simulink model "Proyecto"  (R2023a)
settings: Solver=ode15s  StartTime=0.0  StopTime=10.0  RelTol=1e-3
libraries: fl_lib x16, nesl_utility x6, slpidlib x1
settings Model: Creator=hp  LastModifiedBy=hp
settings DataIOCC: SaveFormat=Array  SaveOutput=off  SignalLogging=off  DSMLogging=off  ReturnWorkspaceOutputs=off  TimeSaveName=t
settings DebuggingCC: AlgebraicLoopMsg=none  MaxConsecutiveZCsMsg=none  ModelReferenceExtraNoncontSigs=none  OperatingPointInterfaceChecksumMismatchMsg=none

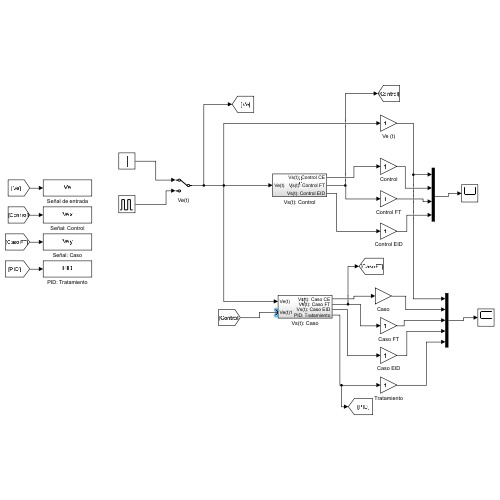
[thumbnail: Simulink's stored preview of the top-level diagram]
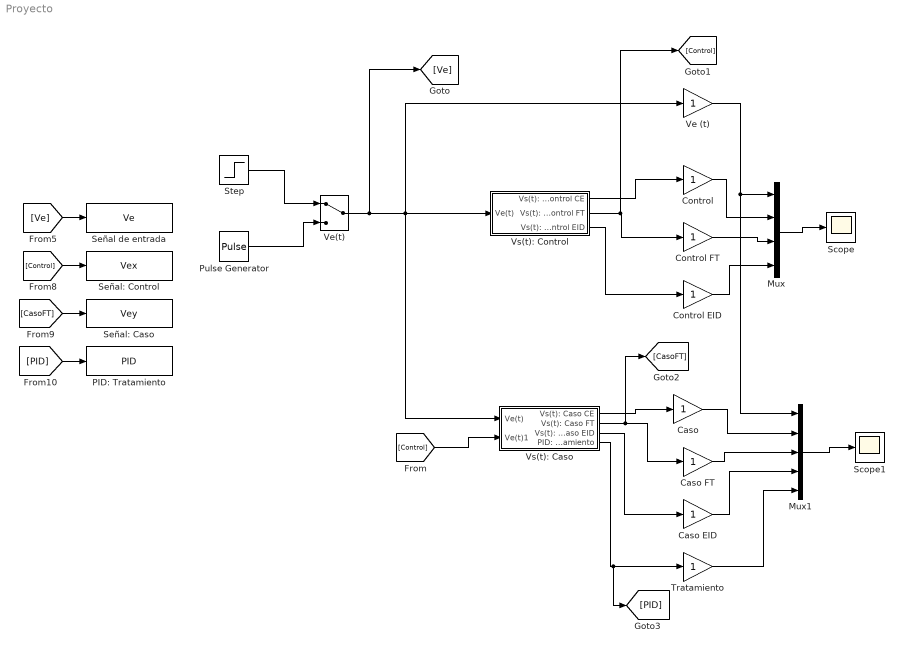
== system Proyecto ==
  Caso : Gain
  Caso EID : Gain
  Caso FT : Gain
  Control : Gain
  Control EID : Gain
  Control FT : Gain
  Mux : Mux
  Mux1 : Mux  Inputs=5
  PID: Tratamiento : ToWorkspace  VariableName=PID  SampleTime=-1
  Pulse Generator : DiscretePulseGenerator  PulseType=Time based  Period=10  PulseWidth=5
  Scope : Scope
  Scope1 : Scope
  Señal de entrada : ToWorkspace  VariableName=Ve  SampleTime=-1
  Señal: Caso : ToWorkspace  VariableName=Vey  SampleTime=-1
  Señal: Control : ToWorkspace  VariableName=Vex  SampleTime=-1
  Step : Step  SampleTime=0
  Tratamiento : Gain
  Ve (t) : Gain
  Ve(t) : ManualSwitch
  Vs(t): Caso : Subsystem
  Vs(t): Control : Subsystem
  wires:
  Step/1 -> Ve(t)/1
  Pulse Generator/1 -> Ve(t)/2
  Ve(t)/1 -> [Ve], Ve (t)/1, Vs(t): Caso/1(Ve(t)), Vs(t): Control/1(Ve(t))
  Mux/1 -> Scope/1
  Ve (t)/1 -> Mux1/1, Mux/1
  Vs(t): Control/1(Vs(t): Control CE) -> Control/1
  Control/1 -> Mux/2
  Vs(t): Caso/1(Vs(t): Caso CE) -> Caso/1
  Vs(t): Control/2(Vs(t): Control FT) -> [Control], Control FT/1
  Caso/1 -> Mux1/2
  Control FT/1 -> Mux/3
  Vs(t): Caso/2(Vs(t): Caso FT) -> [CasoFT], Caso FT/1
  Caso FT/1 -> Mux1/3
  Mux1/1 -> Scope1/1
  Vs(t): Control/3(Vs(t): Control EID) -> Control EID/1
  Control EID/1 -> Mux/4
  Vs(t): Caso/3(Vs(t): Caso EID) -> Caso EID/1
  Caso EID/1 -> Mux1/4
  [Control] -> Señal: Control/1
  [PID] -> PID: Tratamiento/1
  [CasoFT] -> Señal: Caso/1
  [Ve] -> Señal de entrada/1
  [Control] -> Vs(t): Caso/2(Ve(t)1)
  Vs(t): Caso/4(PID: Tratamiento) -> [PID], Tratamiento/1
  Tratamiento/1 -> Mux1/5

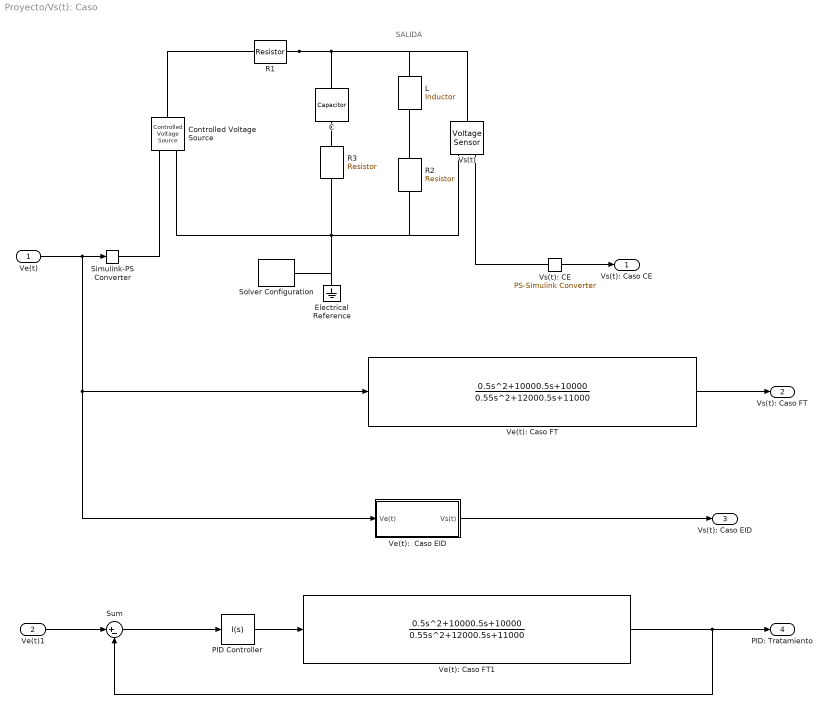
== system Proyecto/Vs(t): Caso ==
  note: SALIDA
  Ve(t) : Inport
  Ve(t)1 : Inport  Port=2
  C : fl_lib/Electrical/Electrical Elements/Capacitor  c=100e-6 F  r=1e-6 Ohm  g=0 1/Ohm  i_specify=off  i_priority=None  i=0 A  i_nominal_specify=off  i_nominal_unit=A  i_nominal_value=1  v_specify=off  v_priority=None  v=0 V  v_nominal_specify=off  v_nominal_unit=V  v_nominal_value=1  vc_specify=off  vc_priority=High  vc=0 V  vc_nominal_specify=off  vc_nominal_unit=V  vc_nominal_value=1
  Controlled Voltage Source : fl_lib/Electrical/Electrical Sources/Controlled Voltage Source
  Electrical Reference : fl_lib/Electrical/Electrical Elements/Electrical Reference
  L : fl_lib/Electrical/Electrical Elements/Inductor  l=500e-3 H  r=0 Ohm  g=1e-9 1/Ohm  i_specify=off  i_priority=None  i=0 A  i_nominal_specify=off  i_nominal_unit=A  i_nominal_value=1  v_specify=off  v_priority=None  v=0 V  v_nominal_specify=off  v_nominal_unit=V  v_nominal_value=1  i_L_specify=off  i_L_priority=High  i_L=0 A  i_L_nominal_specify=off  i_L_nominal_unit=A  i_L_nominal_value=1
  PID Controller : slpidlib/PID Controller  Controller=I  Form=Parallel  TimeDomain=Continuous-time  UseExternalTs=off  SampleTime=-1  IntegratorMethod=Forward Euler  FilterMethod=Forward Euler  ControllerParametersSource=internal  P=0  I=466.911552575517  UseKiTs=off  D=0  N=100  UseFilter=on  TunerSelectOption=Transfer Function Based (PID Tuner App)  InitialConditionSource=internal  InitialConditionForIntegrator=0  InitialConditionForFilter=0  DifferentiatorICPrevScaledInput=0  ExternalReset=none  TrackingMode=off  Kt=1  LimitOutput=off  SatLimitsSource=internal  UpperSaturationLimit=inf  LowerSaturationLimit=-inf  LinearizeAsGain=on  AntiWindupMode=none  Kb=1  LimitIntegrator=off  UpperIntegratorSaturationLimit=inf  LowerIntegratorSaturationLimit=-inf  POutMin=[]  POutMax=[]  IOutMin=[]  IOutMax=[]  DOutMin=[]  DOutMax=[]  NOutMin=[]  NOutMax=[]  SumOutMin=[]  SumOutMax=[]  SaturationOutMin=[]  SaturationOutMax=[]  PParamMin=[]  PParamMax=[]  IParamMin=[]  IParamMax=[]  DParamMin=[]  DParamMax=[]  NParamMin=[]  NParamMax=[]  KbParamMin=[]  KbParamMax=[]  KtParamMin=[]  KtParamMax=[]  KbOutMin=[]  KbOutMax=[]  KtOutMin=[]  KtOutMax=[]  IntegratorOutMin=[]  IntegratorOutMax=[]  FilterOutMin=[]  FilterOutMax=[]  SumI1OutMin=[]  SumI1OutMax=[]  SumI2OutMin=[]  SumI2OutMax=[]  SumI3OutMin=[]  SumI3OutMax=[]  SumI4OutMin=[]  SumI4OutMax=[]  SumDOutMin=[]  SumDOutMax=[]  DifferentiatorOutMin=[]  DifferentiatorOutMax=[]  FilterDiffOutCoefMin=[]  FilterDiffOutCoefMax=[]  ReciprocalOutMin=[]  ReciprocalOutMax=[]  SumDenOutMin=[]  SumDenOutMax=[]  SumNumOutMin=[]  SumNumOutMax=[]  DivideOutMin=[]  DivideOutMax=[]  UdiffTsProdOutMin=[]  UdiffTsProdOutMax=[]  NTsProdOutMin=[]  NTsProdOutMax=[]  UintegralTsProdOutMin=[]  UintegralTsProdOutMax=[]  UngainTsProdOutMin=[]  UngainTsProdOutMax=[]  ClampingZeroOutDataTypeStr=Inherit: Inherit via back propagation  ClampingZeroOutMin=[]  ClampingZeroOutMax=[]  FilterDenConstantOutDataTypeStr=Inherit: Inherit via back propagation  FilterDenConstantOutMin=[]  FilterDenConstantOutMax=[]  PCopyOutDataTypeStr=Inherit: Inherit via back propagation  PCopyOutMin=[]  PCopyOutMax=[]  NCopyOutDataTypeStr=Inherit: Inherit via back propagation  NCopyOutMin=[]  NCopyOutMax=[]  IntegratorContinuousStateAttributes=''  IntegratorStateMustResolveToSignalObject=off  IntegratorRTWStateStorageClass=Auto  FilterContinuousStateAttributes=''  FilterStateMustResolveToSignalObject=off  FilterRTWStateStorageClass=Auto  ParallelPVariant=Disabled  IdealPVariant=Disabled  IVariant=InternalParameters  DVariant=Disabled  IntegratorVariant=Continuous  SatVariant=Disabled  AWVariant=Passthrough  PCopyVariant=Disabled  TRVariant=Disabled  FdbkBlocksVariant=Forward  IdealPFdbkVariant=Disabled  SatFdbkVariant=Disabled  DerivativeFilterVariant=Disabled  NVariant=Disabled  NCopyVariant=Disabled_SignalSpec  FilterICVariant=Disabled  IntegratorICVariant=InternalICs  ExternalResetVariant=Disabled  TRSumVariant=Passthrough  SumFdbkVariant=Disabled  SumVariant=Passthrough_I  TsampFilterVariant=InternalTs  TsampNgainVariant=Passthrough  TsampIntegralVariant=Disabled_SignalSpec  ExternalSaturationOutDataTypeStr=Inherit: Same as second input
  R1 : fl_lib/Electrical/Electrical Elements/Resistor  R=1e3 Ohm  i_specify=off  i_priority=None  i=0 A  i_nominal_specify=off  i_nominal_unit=A  i_nominal_value=1  v_specify=off  v_priority=None  v=0 V  v_nominal_specify=off  v_nominal_unit=V  v_nominal_value=1
  R2 : fl_lib/Electrical/Electrical Elements/Resistor  R=10e3 Ohm  i_specify=off  i_priority=None  i=0 A  i_nominal_specify=off  i_nominal_unit=A  i_nominal_value=1  v_specify=off  v_priority=None  v=0 V  v_nominal_specify=off  v_nominal_unit=V  v_nominal_value=1
  R3 : fl_lib/Electrical/Electrical Elements/Resistor  R=10e3 Ohm  i_specify=off  i_priority=None  i=0 A  i_nominal_specify=off  i_nominal_unit=A  i_nominal_value=1  v_specify=off  v_priority=None  v=0 V  v_nominal_specify=off  v_nominal_unit=V  v_nominal_value=1
  Simulink-PS Converter : nesl_utility/Simulink-PS Converter  PhysicalDomain=network_engine_domain  SubClassName=ps_input  LeftPortType=input  RightPortType=output  PseudoPeriodic=off  Frequencies=[]  NoiseDistribution=none  NoiseParameters=[]  Unit=1  AffineConversion=off  FilteringAndDerivatives=provide  SimscapeFilterOrder=1  InputFilterTimeConstant=0.001  UdotUserProvided=0
  Solver Configuration : nesl_utility/Solver Configuration  PhysicalDomain=network_engine_domain  SubClassName=solver  LeftPortType=input  RightPortType=generic  Tones=[]  Harmonics=[]  SimulateNoise=off  Profile=off  UseLocalSampling=off  EnableSwitchedLinearOptims=on  FrequencyDomain=off  UseCCode=off  RelTol=0.001  AbsTol=0.001  MinStep=1e-09  ToWorkspace=off  RevertToSquareIcSolve=off  NumHomotopyIterations=100  PhasorMode=off  PhasorModeNumHarmonics=1  ConsistencySolver=NEWTON_XTOL_AFTER_FTOL  IndexReductionMethod=DerivativeReplacement  DoDC=off  ResidualTolerance=1e-09  ConsistencyTolSource=GLOBAL  ConsistencyAbsTol=0.001  ConsistencyRelTol=0.001  ConsistencyTolFactor=0.001  UseLocalSolver=off  LocalSolverChoice=NE_BACKWARD_EULER_ADVANCER  ResolveIndetEquations=on  FunctionEvalNumThread=1  LocalSolverSampleTime=0.001  DoFixedCost=off  MaxNonlinIter=3  MaxModeIter=2  ComputeImpulses=off  ImpulseIterations=2  LinearAlgebra=auto  LinearAlgebraNumThread=0  EquationFormulation=NE_TIME_EF  DelaysMemoryBudget=1024  AutomaticFiltering=on  FilteringTimeConstant=0.001  PartitionStorageMethod=AS_NEEDED  PartitionMemoryBudget=1024  PartitionMethod=ROBUST
  Sum : Sum  Inputs=|+-
  Ve(t):  Caso EID : Subsystem
  Ve(t): Caso FT : TransferFcn  Numerator=[0.5, 10000.5, 10000]  Denominator=[0.55, 12000.5, 11000]
  Ve(t): Caso FT1 : TransferFcn  Numerator=[0.5, 10000.5, 10000]  Denominator=[0.55, 12000.5, 11000]
  Vs(t) : fl_lib/Electrical/Electrical Sensors/Voltage Sensor
  Vs(t): CE : nesl_utility/PS-Simulink Converter  PhysicalDomain=network_engine_domain  SubClassName=ps_output  LeftPortType=input  RightPortType=output  PseudoPeriodic=off  Frequencies=[]  VectorFormat=inherit  Unit=inherit  AffineConversion=off
  Vs(t): Caso CE : Outport
  Vs(t): Caso FT : Outport  Port=2
  Vs(t): Caso EID : Outport  Port=3
  PID: Tratamiento : Outport  Port=4
  wires:
  Vs(t): CE/1 -> Vs(t): Caso CE/1
  Ve(t)/1 -> Ve(t): Caso FT/1, Ve(t):  Caso EID/1(Ve(t)), Simulink-PS Converter/1
  Ve(t): Caso FT/1 -> Vs(t): Caso FT/1
  Ve(t):  Caso EID/1(Vs(t)) -> Vs(t): Caso EID/1
  Ve(t): Caso FT1/1 -> Sum/2, PID: Tratamiento/1
  Sum/1 -> PID Controller/1
  Ve(t)1/1 -> Sum/1
  PID Controller/1 -> Ve(t): Caso FT1/1
  connections:
  Controlled Voltage Source/LConn1 -- R1/LConn1
  R1/RConn1 -- L/LConn1 -- Vs(t)/LConn1 -- C/LConn1
  R2/LConn1 -- L/RConn1
  Controlled Voltage Source/RConn2 -- Vs(t)/RConn2 -- R2/RConn1 -- Solver Configuration/RConn1 -- Electrical Reference/LConn1 -- R3/RConn1
  Simulink-PS Converter/RConn1 -- Controlled Voltage Source/RConn1
  Vs(t): CE/LConn1 -- Vs(t)/RConn1
  R3/LConn1 -- C/RConn1

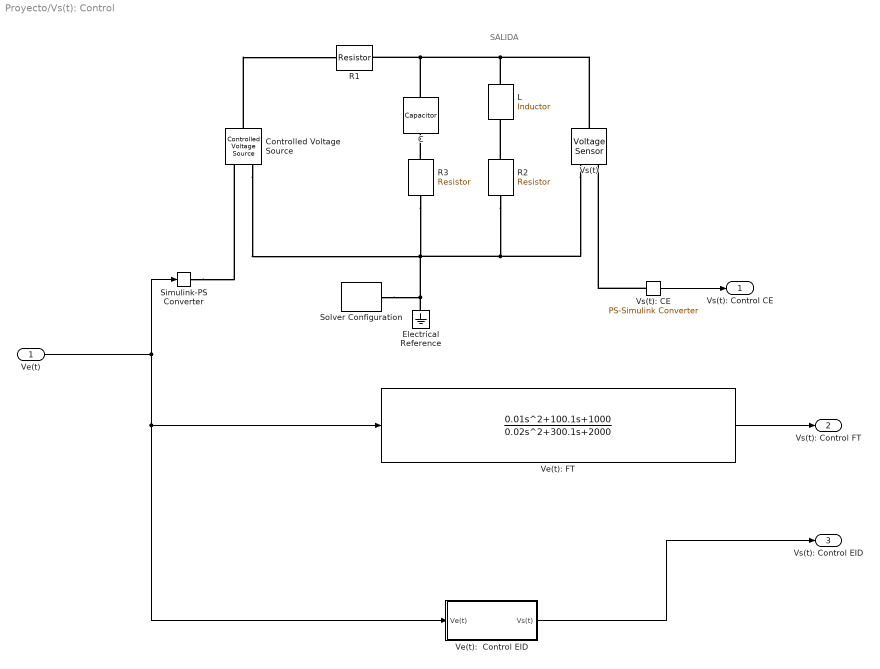
== system Proyecto/Vs(t): Control ==
  note: SALIDA
  Ve(t) : Inport
  C : fl_lib/Electrical/Electrical Elements/Capacitor  c=100e-6 F  r=1e-6 Ohm  g=0 1/Ohm  i_specify=off  i_priority=None  i=0 A  i_nominal_specify=off  i_nominal_unit=A  i_nominal_value=1  v_specify=off  v_priority=None  v=0 V  v_nominal_specify=off  v_nominal_unit=V  v_nominal_value=1  vc_specify=off  vc_priority=High  vc=0 V  vc_nominal_specify=off  vc_nominal_unit=V  vc_nominal_value=1
  Controlled Voltage Source : fl_lib/Electrical/Electrical Sources/Controlled Voltage Source
  Electrical Reference : fl_lib/Electrical/Electrical Elements/Electrical Reference
  L : fl_lib/Electrical/Electrical Elements/Inductor  l=100e-3 H  r=0 Ohm  g=1e-9 1/Ohm  i_specify=off  i_priority=None  i=0 A  i_nominal_specify=off  i_nominal_unit=A  i_nominal_value=1  v_specify=off  v_priority=None  v=0 V  v_nominal_specify=off  v_nominal_unit=V  v_nominal_value=1  i_L_specify=off  i_L_priority=High  i_L=0 A  i_L_nominal_specify=off  i_L_nominal_unit=A  i_L_nominal_value=1
  R1 : fl_lib/Electrical/Electrical Elements/Resistor  R=1e3 Ohm  i_specify=off  i_priority=None  i=0 A  i_nominal_specify=off  i_nominal_unit=A  i_nominal_value=1  v_specify=off  v_priority=None  v=0 V  v_nominal_specify=off  v_nominal_unit=V  v_nominal_value=1
  R2 : fl_lib/Electrical/Electrical Elements/Resistor  R=1e3 Ohm  i_specify=off  i_priority=None  i=0 A  i_nominal_specify=off  i_nominal_unit=A  i_nominal_value=1  v_specify=off  v_priority=None  v=0 V  v_nominal_specify=off  v_nominal_unit=V  v_nominal_value=1
  R3 : fl_lib/Electrical/Electrical Elements/Resistor  R=1e3 Ohm  i_specify=off  i_priority=None  i=0 A  i_nominal_specify=off  i_nominal_unit=A  i_nominal_value=1  v_specify=off  v_priority=None  v=0 V  v_nominal_specify=off  v_nominal_unit=V  v_nominal_value=1
  Simulink-PS Converter : nesl_utility/Simulink-PS Converter  PhysicalDomain=network_engine_domain  SubClassName=ps_input  LeftPortType=input  RightPortType=output  PseudoPeriodic=off  Frequencies=[]  NoiseDistribution=none  NoiseParameters=[]  Unit=1  AffineConversion=off  FilteringAndDerivatives=provide  SimscapeFilterOrder=1  InputFilterTimeConstant=0.001  UdotUserProvided=0
  Solver Configuration : nesl_utility/Solver Configuration  PhysicalDomain=network_engine_domain  SubClassName=solver  LeftPortType=input  RightPortType=generic  Tones=[]  Harmonics=[]  SimulateNoise=off  Profile=off  UseLocalSampling=off  EnableSwitchedLinearOptims=on  FrequencyDomain=off  UseCCode=off  RelTol=0.001  AbsTol=0.001  MinStep=1e-09  ToWorkspace=off  RevertToSquareIcSolve=off  NumHomotopyIterations=100  PhasorMode=off  PhasorModeNumHarmonics=1  ConsistencySolver=NEWTON_XTOL_AFTER_FTOL  IndexReductionMethod=DerivativeReplacement  DoDC=off  ResidualTolerance=1e-09  ConsistencyTolSource=GLOBAL  ConsistencyAbsTol=0.001  ConsistencyRelTol=0.001  ConsistencyTolFactor=0.001  UseLocalSolver=off  LocalSolverChoice=NE_BACKWARD_EULER_ADVANCER  ResolveIndetEquations=on  FunctionEvalNumThread=1  LocalSolverSampleTime=0.001  DoFixedCost=off  MaxNonlinIter=3  MaxModeIter=2  ComputeImpulses=off  ImpulseIterations=2  LinearAlgebra=auto  LinearAlgebraNumThread=0  EquationFormulation=NE_TIME_EF  DelaysMemoryBudget=1024  AutomaticFiltering=on  FilteringTimeConstant=0.001  PartitionStorageMethod=AS_NEEDED  PartitionMemoryBudget=1024  PartitionMethod=ROBUST
  Ve(t):  Control EID : Subsystem
  Ve(t): FT : TransferFcn  Numerator=[0.01, 100.1, 1000]  Denominator=[0.02, 300.1, 2000 ]
  Vs(t) : fl_lib/Electrical/Electrical Sensors/Voltage Sensor
  Vs(t): CE : nesl_utility/PS-Simulink Converter  PhysicalDomain=network_engine_domain  SubClassName=ps_output  LeftPortType=input  RightPortType=output  PseudoPeriodic=off  Frequencies=[]  VectorFormat=inherit  Unit=inherit  AffineConversion=off
  Vs(t): Control CE : Outport
  Vs(t): Control FT : Outport  Port=2
  Vs(t): Control EID : Outport  Port=3
  wires:
  Ve(t)/1 -> Ve(t):  Control EID/1(Ve(t)), Ve(t): FT/1, Simulink-PS Converter/1
  Vs(t): CE/1 -> Vs(t): Control CE/1
  Ve(t): FT/1 -> Vs(t): Control FT/1
  Ve(t):  Control EID/1(Vs(t)) -> Vs(t): Control EID/1
  connections:
  Controlled Voltage Source/LConn1 -- R1/LConn1
  R1/RConn1 -- L/LConn1 -- Vs(t)/LConn1 -- C/LConn1
  R2/LConn1 -- L/RConn1
  Electrical Reference/LConn1 -- Solver Configuration/RConn1 -- Controlled Voltage Source/RConn2 -- R3/RConn1 -- Vs(t)/RConn2 -- R2/RConn1
  Simulink-PS Converter/RConn1 -- Controlled Voltage Source/RConn1
  Vs(t): CE/LConn1 -- Vs(t)/RConn1
  R3/LConn1 -- C/RConn1

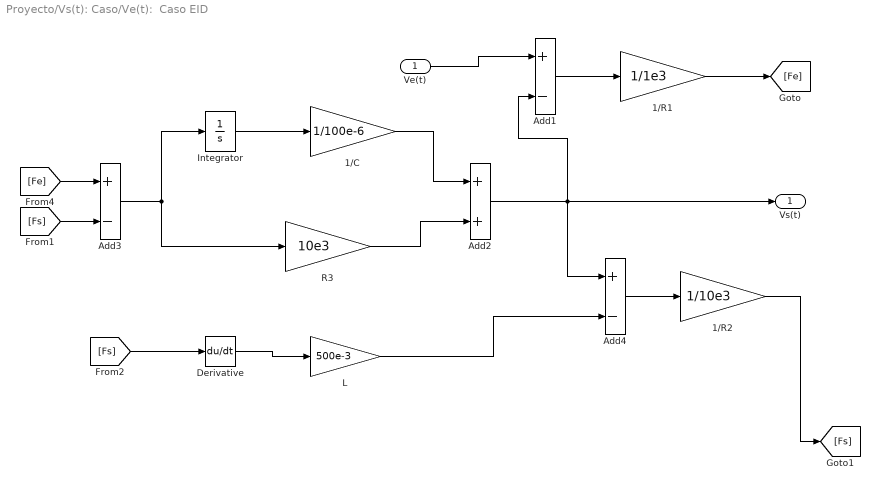
== system Proyecto/Vs(t): Caso/Ve(t):  Caso EID ==
  Ve(t) : Inport
  1/C : Gain  Gain=1/100e-6
  1/R1 : Gain  Gain=1/1e3
  1/R2 : Gain  Gain=1/10e3
  Add1 : Sum  Inputs=+-
  Add2 : Sum
  Add3 : Sum  Inputs=+-
  Add4 : Sum  Inputs=+-
  Derivative : Derivative
  Integrator : Integrator
  L : Gain  Gain=500e-3
  R3 : Gain  Gain=10e3
  Vs(t) : Outport
  wires:
  [Fe] -> Add3/1
  [Fs] -> Add3/2
  Ve(t)/1 -> Add1/1
  Add3/1 -> Integrator/1, R3/1
  Integrator/1 -> 1/C/1
  Derivative/1 -> L/1
  [Fs] -> Derivative/1
  Add1/1 -> 1/R1/1
  1/R1/1 -> [Fe]
  1/R2/1 -> [Fs]
  Add2/1 -> Add4/1, Vs(t)/1, Add1/2
  1/C/1 -> Add2/1
  R3/1 -> Add2/2
  L/1 -> Add4/2
  Add4/1 -> 1/R2/1

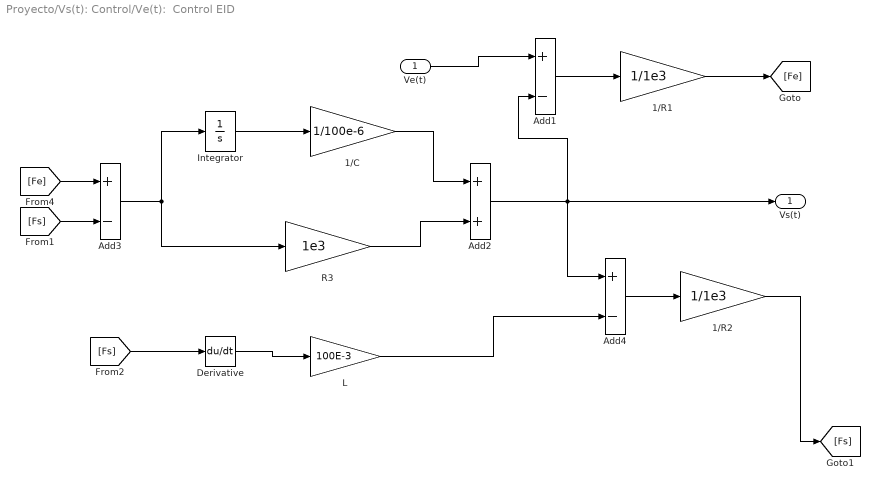
== system Proyecto/Vs(t): Control/Ve(t):  Control EID ==
  Ve(t) : Inport
  1/C : Gain  Gain=1/100e-6
  1/R1 : Gain  Gain=1/1e3
  1/R2 : Gain  Gain=1/1e3
  Add1 : Sum  Inputs=+-
  Add2 : Sum
  Add3 : Sum  Inputs=+-
  Add4 : Sum  Inputs=+-
  Derivative : Derivative
  Integrator : Integrator
  L : Gain  Gain=100E-3
  R3 : Gain  Gain=1e3
  Vs(t) : Outport
  wires:
  [Fe] -> Add3/1
  [Fs] -> Add3/2
  Ve(t)/1 -> Add1/1
  Add3/1 -> Integrator/1, R3/1
  Integrator/1 -> 1/C/1
  Derivative/1 -> L/1
  [Fs] -> Derivative/1
  Add1/1 -> 1/R1/1
  1/R1/1 -> [Fe]
  1/R2/1 -> [Fs]
  Add2/1 -> Add4/1, Vs(t)/1, Add1/2
  1/C/1 -> Add2/1
  R3/1 -> Add2/2
  L/1 -> Add4/2
  Add4/1 -> 1/R2/1
